simulink model "RKTI"  (R2024b)
settings: Solver=FixedStepAuto  StartTime=0.0  StopTime=10.0  RelTol=1e-3
undefined symbols (not defined in the file): B_TI_MAN, KRKTE, TEMIN, TI_MAN, TI_MAN_START_MX
settings Model: Creator=Student  LastModifiedBy=Student
settings OptimizationCC: DefaultParameterBehavior=Inlined  EnhancedBackFolding=on  PassReuseOutputArgsAs=Individual arguments  ZeroExternalMemoryAtStartup=off  ZeroInternalMemoryAtStartup=off  OptimizeBlockOrder=speed  DifferentSizesBufferReuse=on  OptimizationCustomize=off  EfficientTunableParamExpr=on
settings DebuggingCC: ParameterTunabilityLossMsg=error  SFUnexpectedBacktrackingDiag=warning  SFNoUnconditionalDefaultTransitionDiag=warning
settings HardwareCC: TargetBitPerPointer=64  TargetBitPerSizeT=64  TargetBitPerPtrDiffT=64  TargetLongLongMode=on  TargetIntDivRoundTo=Zero  TargetEndianess=LittleEndian  TargetWordSize=64  TargetHWDeviceType=MATLAB Host  ProdEqTarget=off
settings ModelReferenceCC: EnableRefExpFcnMdlSchedulingChecks=on
settings SFSimCC: MATLABDynamicMemAlloc=off
settings RTWCC: Description=Embedded Coder  SystemTargetFile=ert.tlc  GenCodeOnly=on  TemplateMakefile=ert_default_tmf  GenerateReport=on  BuildConfiguration=Debug  LaunchReport=on  GPUComputeCapability=3.5
settings CodeAppCC: ForceParamTrailComments=on  IgnoreCustomStorageClasses=off  OperatorAnnotations=on  SimulinkDataObjDesc=on  SFDataObjDesc=on  InsertBlockDesc=on  EnableCustomComments=on
settings ERTTargetCC: TargetLangStandard=C99 (ISO)  GenerateSampleERTMain=on  ERTCustomFileTemplate=example_file_process.tlc

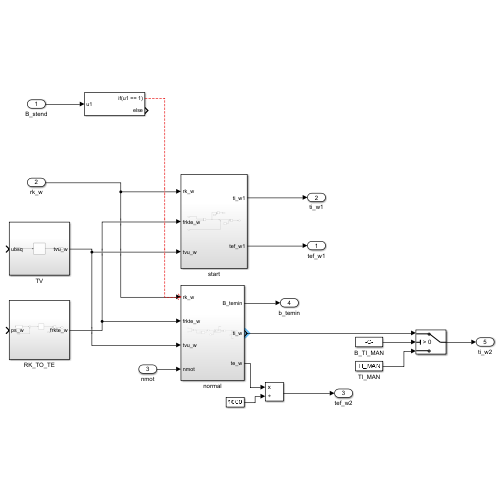
[thumbnail: Simulink's stored preview of the top-level diagram]
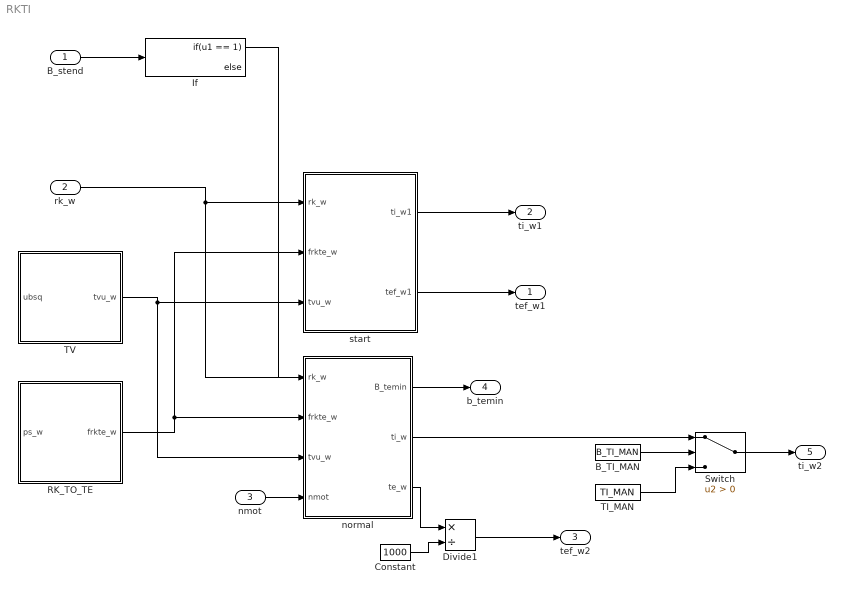
== system RKTI ==
  B_stend : Inport  OutDataTypeStr=boolean
  rk_w : Inport  Port=2  OutDataTypeStr=fixdt(0,8,16/256,0)
  nmot : Inport  Port=3
  B_TI_MAN : Constant  Value=B_TI_MAN  OutDataTypeStr=boolean
  Constant : Constant  Value=1000
  Divide1 : Product  Inputs=*/  OutMin=[0]  OutMax=[1.04854]  OutDataTypeStr=fixdt(0,16,1.04856/65536,0)  SaturateOnIntegerOverflow=on
  If : If  IfExpression=u1 == 1
  RK_TO_TE : Subsystem
  Switch : Switch  Criteria=u2 > Threshold  SaturateOnIntegerOverflow=off  InputSameDT=off
  TI_MAN : Constant  Value=TI_MAN  OutMin=[0]  OutMax=[1048.54]  OutDataTypeStr=fixdt(0,16,1048.56/65536,0)
  TV : Subsystem
  normal : Subsystem
  start : Subsystem
  tef_w1 : Outport  OutMin=[0]  OutMax=[1.04854]  OutDataTypeStr=fixdt(0,16,1.04856/65536,0)
  ti_w1 : Outport  Port=2  OutMin=[0]  OutMax=[1048.54]  OutDataTypeStr=fixdt(0,16,1048.56/65536,0)
  tef_w2 : Outport  Port=3  OutMin=[0]  OutMax=[1.04854]  OutDataTypeStr=fixdt(0,16,1.04856/65536,0)
  b_temin : Outport  Port=4
  ti_w2 : Outport  Port=5  OutMin=[0]  OutMax=[1048.54]  OutDataTypeStr=fixdt(0,16,1048.56/65536,0)
  wires:
  B_stend/1 -> If/1
  If/1 -> ?
  rk_w/1 -> start/1(rk_w), normal/1(rk_w)
  Constant/1 -> Divide1/2
  Divide1/1 -> tef_w2/1
  TV/1(tvu_w) -> normal/3(tvu_w), start/3(tvu_w)
  RK_TO_TE/1(frkte_w) -> start/2(frkte_w), normal/2(frkte_w)
  normal/2(ti_w) -> Switch/1
  B_TI_MAN/1 -> Switch/2
  TI_MAN/1 -> Switch/3
  start/1(ti_w1) -> ti_w1/1
  start/2(tef_w1) -> tef_w1/1
  normal/1(B_temin) -> b_temin/1
  normal/3(te_w) -> Divide1/1
  Switch/1 -> ti_w2/1
  nmot/1 -> normal/4(nmot)

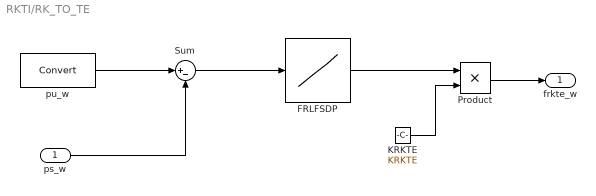
== system RKTI/RK_TO_TE ==
  ps_w : Inport
  FRLFSDP : Lookup_n-D  NumberOfTableDimensions=1  BreakpointsForDimension1=[0 100 200 300 400 500 600 700 800 900 1000]  Table=[1 0.986022 0.972595 0.959716 0.947326 0.935424 0.92395 9.128723000000001 9.021910999999999 8.918761999999999 8.819274]  ExtrapMethod=Clip  InternalRulePriority=Speed  OutDataTypeStr=fixdt(1,16,2^-8,0)  RndMeth=Simplest  LockScale=on
  KRKTE : Constant  Value=KRKTE  OutMin=[0]  OutMax=[8.73787]  OutDataTypeStr=fixdt(0,16,8.738/65536,0)
  Product : Product  OutMin=[0]  OutMax=[8.73787]  OutDataTypeStr=fixdt(0,16,8.738/65536,0)  SaturateOnIntegerOverflow=on
  Sum : Sum  Inputs=|+-
  pu_w : DataTypeConversion  SaturateOnIntegerOverflow=off  RndMeth=Floor
  frkte_w : Outport  OutMin=[0]  OutMax=[8.73787]  OutDataTypeStr=fixdt(0,16,8.738/65536,0)
  wires:
  ps_w/1 -> Sum/2
  pu_w/1 -> Sum/1
  Sum/1 -> FRLFSDP/1
  FRLFSDP/1 -> Product/1
  KRKTE/1 -> Product/2
  Product/1 -> frkte_w/1

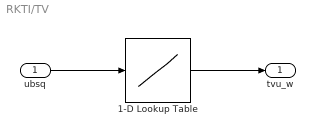
== system RKTI/TV ==
  ubsq : Inport
  1-D Lookup Table : Lookup_n-D  NumberOfTableDimensions=1  BreakpointsForDimension1=[6;8;10.5;12.5;15.2]  Table=[11.712;7.952;4;1.504;0.608]  ExtrapMethod=Clip  InternalRulePriority=Speed  RndMeth=Simplest
  tvu_w : Outport
  wires:
  1-D Lookup Table/1 -> tvu_w/1
  ubsq/1 -> 1-D Lookup Table/1

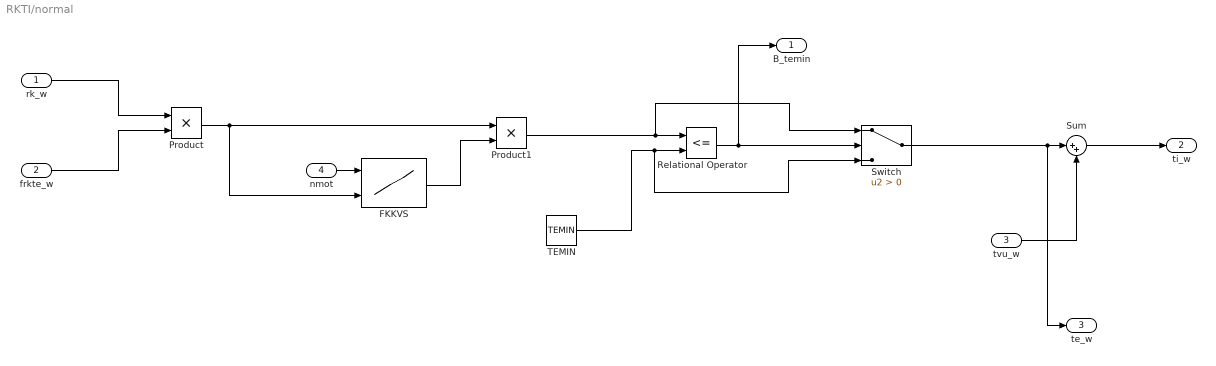
== system RKTI/normal ==
  rk_w : Inport
  frkte_w : Inport  Port=2  OutMin=[0]  OutMax=[8.73787]  OutDataTypeStr=fixdt(0,16,8.738/65536,0)
  tvu_w : Inport  Port=3  OutMin=[0]  OutMax=[1048.54]  OutDataTypeStr=fixdt(0,16,1048.56/65536,0)
  nmot : Inport  Port=4
  FKKVS : Lookup_n-D  BreakpointsForDimension1=[720;800;1000;1200;1520;1760;2000;2240;2520;3000;3520;4000;4520;5200;5800;6400;7000;7600;8200;8800]  BreakpointsForDimension2=[9.007999999999999;13.008;18;24;30;36;42;48;54;60;66;72;78;84;90;100;110;120;130;140]  Table=[1 1 1 1 1 1 1 1 1 1 1 1 1 1 1 1 1 1 1 1;1 1 1 1 1 1 1 1 1 1 1 1 1 1 1 1 1 1 1 1;0.950012 0.950012 1 1.029998 1.029998 1.019989 1.019989 1 1 1 1 1 1 1 1 1 1 1 1 1;1 0.950012 1 1.029998 1.029998 1.019989 1.019989 1 1 1 1 1 1 1 1 1 1 1 1 1;1 1 1 1.029998 1.02998 1.019989 1.019989 1 1 1 1 1 1 1 1 1 1 1 1 1;1 1 1 1 1 1 1 1 1 1 1 1 1 1 1 1 1 1 1 1;1 1 1 1 1 1 1 1 1.010009 1.010009 1.010009 1.010009 1.010009 1.010009 1.010009 1.010009 1.010009 1.010009 1.010009 1.010009;1 1 1 1 1 1 1 1 1.010009 1.010009 1.010009 1.010009 1.010009 1.010009 1.010009 1.010009 1.010009 1.010009 1.010009 1.010009;1 1 1 1 1 1 1 1 1.049987 1.040008 1.040008 1.040008 1.040008 1.040008 1.040008 1.040008 1.040008 1.040008 1.040008 1.040008;1 1 1 1 1 1 1 1.019989 1.010009 1.010009 1.040008 1.040008 1.040008 1.040008 1.040008 1.040008 1.040008 1.040008 1.040008 1.040008;1 1 1 1 1 1 1 1.049987 1.040008 1.040008 1.019989 1.019989 1.019989 1.019989 1.019989 1.019989 1.019989 1.019989 1.019989 1.019989;1 1 1 1 1 1.010009 1.010009 1.019989 1.010009 1 1.010009 1.010009 1.010009 1.010009 1.010009 1.010009 1.010009 1.010009 1.010009 1.010009;1 1 1 9.800109000000001 1 1 1 1 1 1 1 1 1 1 1 1 1 1 1 1;1 1 1 1 1.029998 1.010009 1.010009 1.029998 1.029998 1 1 1 1.019989 1.010009 1.010009 1.010009 1.010009 1.010009 1.010009 1.010009;1 1 1 1 1.019989 1.019989 1.029998 1.029998 1.029998 1.010009 1.010009 1.010009 1.010009 1.010009 1.010009 1.010009 1.010009 1.010009 1.010009 1.010009;1 1 1 1 1.019989 1.019989 1.029998 1.029998 1.029998 1.010009 1.010009 1.010009 1.010009 1.010009 1.010009 1.010009 1.010009 1.010009 1.010009 1.010009;1 1 1 1 1 1 1 1 1 1 1 1 1 1 1 1 1 1 1 1;1 1 1 1 1 1 1 1 1 1 1 1 1 1 1 1 1 1 1 1;1 1 1 1 1 1 1 1 1 1 1 1 1 1 1 1 1 1 1 1;1 1 1 1 1 1 1 1 1 1 1 1 1 1 1 1 1 1 1 1]  ExtrapMethod=Clip  InternalRulePriority=Speed  RndMeth=Simplest
      settings: InputPortMap=u0,u1
  Product : Product
  Product1 : Product
  Relational Operator : RelationalOperator  Operator=<=  OutDataTypeStr=boolean  RndMeth=Simplest  InputSameDT=off
  Sum : Sum  Inputs=|++  OutMin=[0]  OutMax=[1048.54]  OutDataTypeStr=fixdt(0,16,1048.56/65536,0)  SaturateOnIntegerOverflow=on
  Switch : Switch  Criteria=u2 > Threshold  OutMin=[0]  OutMax=[1048.54]  OutDataTypeStr=fixdt(0,16,1048.56/65536,0)  InputSameDT=off
  TEMIN : Constant  Value=TEMIN  OutMin=[0]  OutMax=[1048.54]  OutDataTypeStr=fixdt(0,16,1048.56/65536,0)
  B_temin : Outport  OutMin=[0]  OutMax=[1]  OutDataTypeStr=boolean
  ti_w : Outport  Port=2  OutMin=[0]  OutMax=[1048.54]  OutDataTypeStr=fixdt(0,16,1048.56/65536,0)
  te_w : Outport  Port=3  OutMin=[0]  OutMax=[1048.54]  OutDataTypeStr=fixdt(0,16,1048.56/65536,0)
  wires:
  rk_w/1 -> Product/1
  frkte_w/1 -> Product/2
  Product/1 -> FKKVS/2, Product1/1
  nmot/1 -> FKKVS/1
  FKKVS/1 -> Product1/2
  Product1/1 -> Switch/1, Relational Operator/1
  TEMIN/1 -> Switch/3, Relational Operator/2
  Relational Operator/1 -> B_temin/1, Switch/2
  Switch/1 -> te_w/1, Sum/1
  tvu_w/1 -> Sum/2
  Sum/1 -> ti_w/1

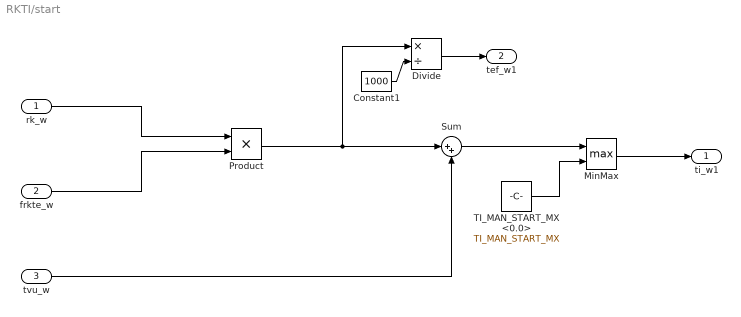
== system RKTI/start ==
  rk_w : Inport
  frkte_w : Inport  Port=2  OutMin=[0]  OutMax=[8.73787]  OutDataTypeStr=fixdt(0,16,8.738/65536,0)
  tvu_w : Inport  Port=3  OutMin=[0]  OutMax=[1048.54]  OutDataTypeStr=fixdt(0,16,1048.56/65536,0)
  Constant1 : Constant  Value=1000
  Divide : Product  Inputs=*/  OutMin=[0]  OutMax=[1.04854]  OutDataTypeStr=fixdt(0,16,1.04856/65536,0)  SaturateOnIntegerOverflow=on
  MinMax : MinMax  Function=max  Inputs=2  OutMin=[0]  OutMax=[1048.54]  OutDataTypeStr=fixdt(0,16,1048.56/65536,0)  SaturateOnIntegerOverflow=on
  Product : Product
  Sum : Sum  Inputs=|++
  TI_MAN_START_MX <0.0> : Constant  Value=TI_MAN_START_MX  OutMin=[0]  OutMax=[1048.54]  OutDataTypeStr=fixdt(0,16,1048.56/65536,0)
  ti_w1 : Outport  OutMin=[0]  OutMax=[1048.54]  OutDataTypeStr=fixdt(0,16,1048.56/65536,0)
  tef_w1 : Outport  Port=2  OutMin=[0]  OutMax=[1.04854]  OutDataTypeStr=fixdt(0,16,1.04856/65536,0)
  wires:
  rk_w/1 -> Product/1
  frkte_w/1 -> Product/2
  Product/1 -> Sum/1, Divide/1
  Constant1/1 -> Divide/2
  tvu_w/1 -> Sum/2
  TI_MAN_START_MX <0.0>/1 -> MinMax/2
  Sum/1 -> MinMax/1
  MinMax/1 -> ti_w1/1
  Divide/1 -> tef_w1/1
